simulink model "ADAS_Overtaking_T2_BlockedSides"  (R2024b)
settings: Solver=FixedStepDiscrete  StartTime=0.0  StopTime=40  FixedStep=0.1  RelTol=1e-3
undefined symbols (not defined in the file): DiscIntNeverNeededParam
libraries: simulink x1
settings Model: Creator=chikc  LastModifiedBy=chikc

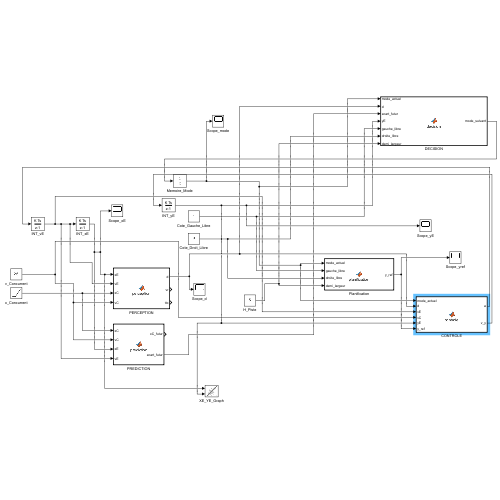
[thumbnail: Simulink's stored preview of the top-level diagram]
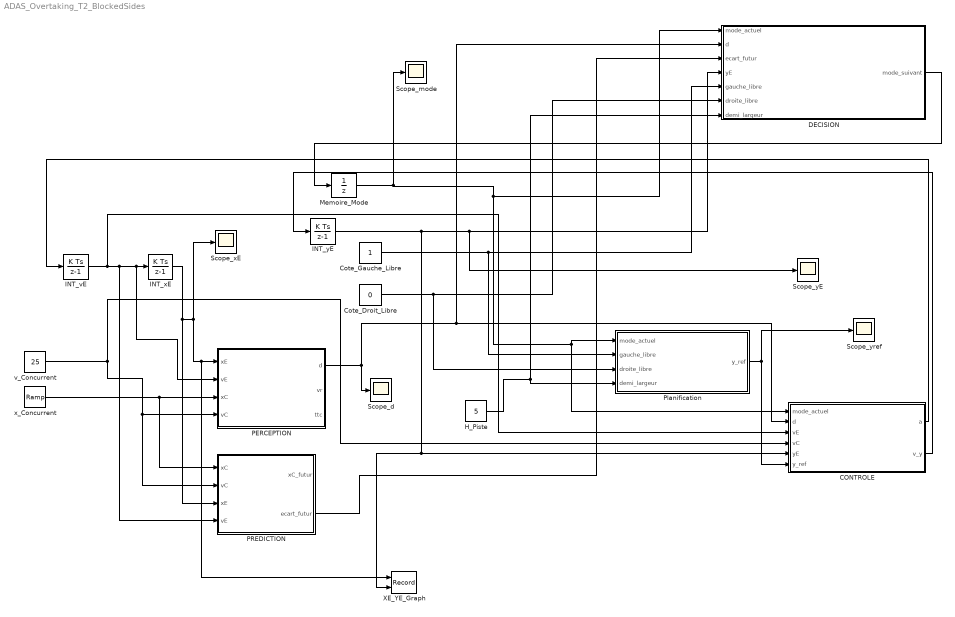
== system ADAS_Overtaking_T2_BlockedSides ==
  " x_Concurrent " : simulink/Sources/Ramp  slope=25  start=0  InitialOutput=100
  CONTROLE : MATLAB Function  TreatAsAtomicUnit=on
  Cote_Droit_Libre : Constant  Value=0
  Cote_Gauche_Libre : Constant
  DECISION : MATLAB Function  TreatAsAtomicUnit=on
  H_Piste : Constant  Value=5
  INT_vE : DiscreteIntegrator  InitialCondition=30  SampleTime=0.1  ICPrevOutput=DiscIntNeverNeededParam  ICPrevScaledInput=DiscIntNeverNeededParam
  INT_xE : DiscreteIntegrator  SampleTime=0.1  ICPrevOutput=DiscIntNeverNeededParam  ICPrevScaledInput=DiscIntNeverNeededParam
  INT_yE : DiscreteIntegrator  SampleTime=0.1  ICPrevOutput=DiscIntNeverNeededParam  ICPrevScaledInput=DiscIntNeverNeededParam
  Memoire_Mode : UnitDelay  SampleTime=0.1  HasFrameUpgradeWarning=on
  PERCEPTION : MATLAB Function  TreatAsAtomicUnit=on
  PREDICTION : MATLAB Function  TreatAsAtomicUnit=on
  Planification : MATLAB Function  TreatAsAtomicUnit=on
  Scope_d : Scope
  Scope_mode : Scope
  Scope_xE : Scope
  Scope_yE : Scope
  Scope_yref : Scope
  XE_YE_Graph : Record  FileSettingsInternal="{\"entries\":[{\"content\":{\"excelSettings\":{\"content\":{},\"type\":\"Streamout.ExcelSettings\"}},\"type\":\"Streamout.FileSettingStorage\",\"uuid\":\"\"}],\"packageUris\":[\"http:\\/\\/schema.mathworks.com\\/mf0\\/streamout_blocks\\/R2020a\"],\"version\":\"1.0\"}"  Layout=[1 1]  SignalsInternal="{\"entries\":[{\"content\":{\"signals\":[{\"content\":{\"blockPath\":[],\"dimensions\":[1],\"domain\":\"\",\"lineColor\":\"#a2142f\",\"plots\":[ 1 ],\"port\":1,\"signalID\":1,\"signalName\":\"INT_xE\"},\"type\":\"RecordBlkView.Signal\",\"uuid\":\"\"},{\"content\":{\"blockPath\":[],\"dimensions\":[1],\"domain\":\"\",\"lineColor\":\"#139fff\",\"plots\":[ 1 ],\"port\":2,\"signalID\":2,\"signalName\":\"INT_yE\"},\"type\":\"RecordBlkView.Signal\",\"uuid\":\"\"}]},\"type\":\"RecordBlkView.InputSignals\",\"uuid\":\"\"}],\"packageUris\":[\"http:\\/\\/schema.mathworks.com\\/mf0\\/streamout_blocks\\/R2020a\"],\"version\":\"1.0\"}"  VisualizationBindings="{\"xyplotplugin\":{\"info\":[{\"series\":[{\"bindingParametersList\":[{\"parameter\":\"X-Axis\",\"signalID\":1,\"signalName\":\"INT_xE\"},{\"parameter\":\"Y-Axis\",\"signalID\":2,\"signalName\":\"INT_yE\"}],\"seriesID\":0}],\"subplotID\":1}]}}"  CompatibilityTag=XY
  v_Concurrent : Constant  Value=25
  wires:
  INT_vE/1 -> CONTROLE/3(vE), PREDICTION/4(vE), PERCEPTION/2(vE), INT_xE/1
  " x_Concurrent "/1 -> PREDICTION/1(xC), PERCEPTION/3(xC)
  v_Concurrent/1 -> CONTROLE/4(vC), PREDICTION/2(vC), PERCEPTION/4(vC)
  Memoire_Mode/1 -> CONTROLE/1(mode_actuel), Planification/1(mode_actuel), DECISION/1(mode_actuel), Scope_mode/1
  DECISION/1(mode_suivant) -> Memoire_Mode/1
  PERCEPTION/1(d) -> CONTROLE/2(d), DECISION/2(d), Scope_d/1
  PREDICTION/2(ecart_futur) -> DECISION/3(ecart_futur)
  INT_yE/1 -> CONTROLE/5(yE), XE_YE_Graph/2, Scope_yE/1, DECISION/4(yE)
  Cote_Gauche_Libre/1 -> Planification/2(gauche_libre), DECISION/5(gauche_libre)
  Cote_Droit_Libre/1 -> DECISION/6(droite_libre), Planification/3(droite_libre)
  H_Piste/1 -> DECISION/7(demi_largeur), Planification/4(demi_largeur)
  Planification/1(y_ref) -> Scope_yref/1, CONTROLE/6(y_ref)
  CONTROLE/1(a) -> INT_vE/1
  CONTROLE/2(v_y) -> INT_yE/1
  INT_xE/1 -> PREDICTION/3(xE), Scope_xE/1, XE_YE_Graph/1, PERCEPTION/1(xE)

== matlab function ADAS_Overtaking_T2_BlockedSides/PREDICTION ==
  data: xC input; xC_futur output; vC input; xE input; vE input; ecart_futur output
function [xC_futur, ecart_futur] = prediction(xC, vC, xE, vE)
% Constant-speed prediction over a 2 s horizon.
Tp = 2.0;                     % prediction horizon (s)
xC_futur = xC + vC*Tp;        % m
xE_futur = xE + vE*Tp;        % m, assuming constant ego speed
ecart_futur = xC_futur - xE_futur;
end

== matlab function ADAS_Overtaking_T2_BlockedSides/PERCEPTION ==
  data: xE input; d output; vE input; xC input; vC input; vr output; ttc output
function [d, vr, ttc] = perception(xE, vE, xC, vC)
% Relative position and speed from simulated vehicle states.
% d > 0: target ahead; d < 0: ego vehicle ahead.
d = xC - xE;      % m
vr = vE - vC;     % m/s, closing speed
if (d > 0) && (vr > 0.001)
    ttc = d / vr; % s, assuming constant speeds
else
    ttc = 1.0e6;  % sentinel value when positive TTC is undefined
end
end

== matlab function ADAS_Overtaking_T2_BlockedSides/DECISION ==
  data: mode_actuel input; mode_suivant output; d input; ecart_futur input; yE input; gauche_libre input; droite_libre input; demi_largeur input

function mode_suivant = decision(mode_actuel, d, ecart_futur, ...
    yE, gauche_libre, droite_libre, demi_largeur)

% Modes:
% 0 = FOLLOW
% 1 = OVERTAKE
% 2 = RETURN
% 3 = FINISHED

% Keep the current mode unless a transition condition is met.
mode_suivant = mode_actuel;

marge_bord = 1.5;
y_pass = 3.0;

piste_ok = (demi_largeur >= abs(y_pass) + marge_bord);

cote_disponible = (gauche_libre > 0.5) || ...
                  (droite_libre > 0.5);

if mode_actuel == 0
    if (d <= 60.0) && (d > 20.0) && ...
       (ecart_futur > 15.0) && ...
       piste_ok && cote_disponible

        mode_suivant = 1;
    end

elseif mode_actuel == 1
    if d <= -15.0
        mode_suivant = 2;
    end

elseif mode_actuel == 2
    if abs(yE) < 0.15
        mode_suivant = 3;
    end

else
    mode_suivant = 3;
end

end

== matlab function ADAS_Overtaking_T2_BlockedSides/Planification ==
  data: mode_actuel input; y_ref output; gauche_libre input; droite_libre input; demi_largeur input
function y_ref = planification(mode_actuel, gauche_libre, ...
    droite_libre, demi_largeur)
% Choose a fixed lateral offset when overtaking is allowed.
y_ref = 0.0;
y_pass = 3.0;
piste_ok = (demi_largeur >= y_pass + 1.5);
if mode_actuel == 1 && piste_ok
    if gauche_libre > 0.5
        y_ref = y_pass;
    elseif droite_libre > 0.5
        y_ref = -y_pass;
    end
end
end

== matlab function ADAS_Overtaking_T2_BlockedSides/CONTROLE ==
  data: mode_actuel input; a output; d input; vE input; vC input; yE input; y_ref input; v_y output
function [a, v_y] = controle(mode_actuel, d, vE, vC, yE, y_ref)
% Proportional longitudinal and lateral control.
% Outputs are acceleration and lateral speed.
% The model does not calculate a steering angle.
v_libre = 30.0; % m/s
if mode_actuel == 0  % following mode: adapt speed to the gap
    d_ref = 20.0;  % m, desired following gap
    v_dem = vC + 0.35*(d - d_ref);
    v_dem = min(v_libre,max(0.0,v_dem));
else
    v_dem = v_libre;
end
% Proportional acceleration command limited to [-4, 3] m/s^2.
a_non_lim = 1.5*(v_dem - vE);
a = min(3.0,max(-4.0,a_non_lim));
% Proportional lateral speed command limited to +/-1.2 m/s.
v_y_non_lim = 0.8*(y_ref - yE);
v_y = min(1.2,max(-1.2,v_y_non_lim));
end
